simulink model "netra_dist"  (R2026b)
settings: Solver=VariableStepAuto  StopTime=14400
values from neighbouring files (symbols this model uses):
  m = 'netra_dist'; if bdIsLoaded(m), close_system(m,0); end    [build_district_sim.m]    (also in run_district_sim.m = @(x) mean(x,'omitnan'))
  n = numel(arr)    [run_district_sim.m]
settings Model: Creator=dron  LastModifiedBy=dron

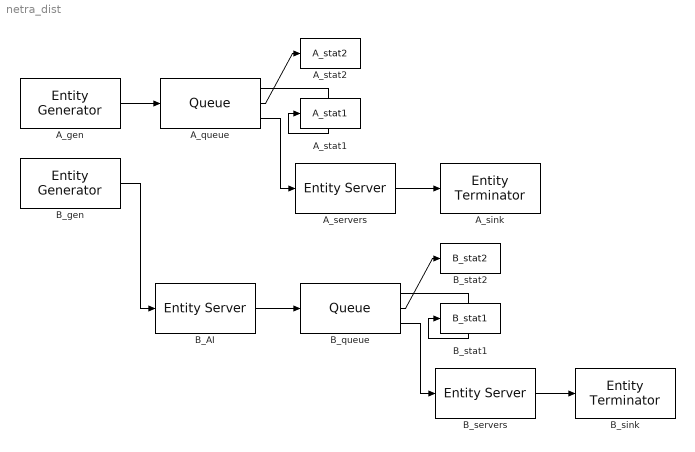
== system netra_dist ==
  A_gen : EntityGenerator  OutputPortMessageModes=m  TimeSource=MATLAB action  IntergenerationTimeAction=dt = -log(rand)*2.4;  EntityType=Structured  EntityTypeName=Entity
  A_queue : Queue  InputPortMessageModes=m  OutputPortMessageModes=n,n,m  Capacity=1e6  NumberEntitiesInBlock=on  AverageWait=on
      settings: OutputPortMap=o1,o2,o5
  A_servers : EntityServer  InputPortMessageModes=m  OutputPortMessageModes=m  Capacity=2  ServiceTimeSource=MATLAB action  ServiceTimeAction=dt = -log(rand)*10;
  A_sink : EntityTerminator  InputPortMessageModes=m
  A_stat1 : ToWorkspace  VariableName=A_stat1  SaveFormat=Timeseries  SampleTime=-1
  A_stat2 : ToWorkspace  VariableName=A_stat2  SaveFormat=Timeseries  SampleTime=-1
  B_AI : EntityServer  InputPortMessageModes=m  OutputPortMessageModes=m  Capacity=1000  ServiceTimeValue=1
  B_gen : EntityGenerator  OutputPortMessageModes=m  TimeSource=MATLAB action  IntergenerationTimeAction=dt = -log(rand)*6.13613;  GenerateAction=u=rand; g=2+(u>0.612777)+(u>0.801435); entity.Grade=g+1;  AttributeName=Grade  EntityType=Structured  EntityTypeName=PatientB
  B_queue : Queue  InputPortMessageModes=m  OutputPortMessageModes=n,n,m  Capacity=1e6  QueueType=Priority  PrioritySource=Grade  SortingDirection=Descending  NumberEntitiesInBlock=on  AverageWait=on
      settings: OutputPortMap=o1,o2,o5
  B_servers : EntityServer  InputPortMessageModes=m  OutputPortMessageModes=m  Capacity=2  ServiceTimeSource=MATLAB action  ServiceTimeAction=dt = -log(rand)*10;
  B_sink : EntityTerminator  InputPortMessageModes=m
  B_stat1 : ToWorkspace  VariableName=B_stat1  SaveFormat=Timeseries  SampleTime=-1
  B_stat2 : ToWorkspace  VariableName=B_stat2  SaveFormat=Timeseries  SampleTime=-1
  wires:
  B_queue/3 -> B_servers/1
  B_queue/1 -> B_stat1/1
  B_queue/2 -> B_stat2/1
  B_servers/1 -> B_sink/1
  A_servers/1 -> A_sink/1
  B_AI/1 -> B_queue/1
  A_queue/1 -> A_stat1/1
  A_queue/3 -> A_servers/1
  A_queue/2 -> A_stat2/1
  B_gen/1 -> B_AI/1
  A_gen/1 -> A_queue/1
